simulink model "b0_loop"  (R2023b)
settings: Solver=FixedStepDiscrete  StartTime=0.0  StopTime=60  FixedStep=0.001  RelTol=1e-3
undefined symbols (not defined in the file or in its folder): DiscIntNeverNeededParam
settings Model: Creator=28447  LastModifiedBy=28447
settings SFSimCC: SimCustomHeaderCode=extern void b0_ident_sim(float iq, float u, float omega, float e1, float v, float *b0, float *du);  SimUserIncludeDirs=D:\Desktop\RCESO\simulink
settings SFSimCC: SimUserSources=|
  | D:\Desktop\RCESO\simulink\b0_ident.c
  | D:\Desktop\RCESO\simulink\b0_ident_wrap.c

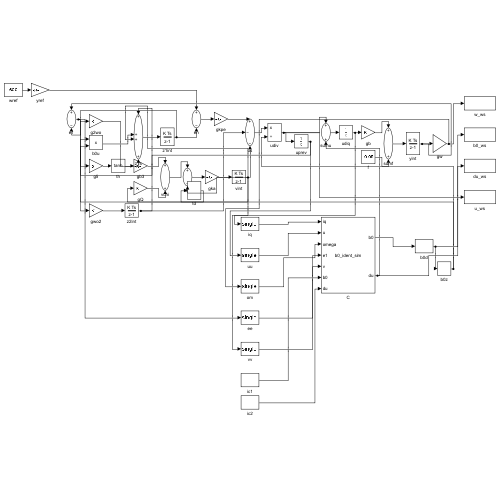
[thumbnail: Simulink's stored preview of the top-level diagram]
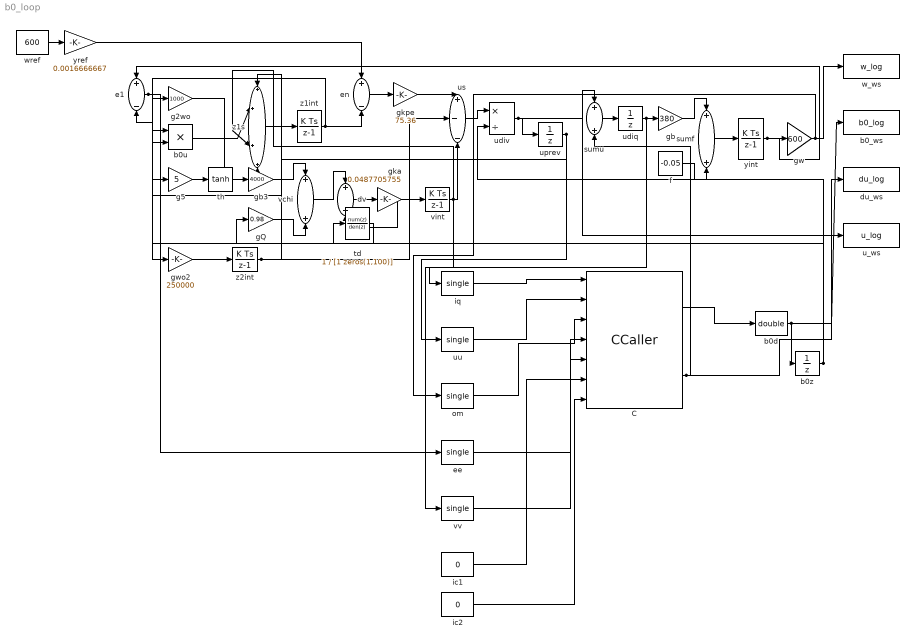
== system b0_loop ==
  C : CCaller  FunctionName=b0_ident_sim  PortSpecificationStruct="%)30     .    ^ L   8    (     @         %    \"     <    !     0         %  0 \"0    $    _    07)G3F%M90  4&]R=$YA;64 4V-O<&4     26YD97@     5'EP90      4VEZ90      27-';&]B86P   X    P    !@    @    $          4    (     0    (    !         !   @!I<0  #@   #     &    \"     0         !0    @    !     @    $         $  \" &EQ   .    .     8    (    !          %    \"     $    %     0         0  ...(+3754 chars)"
  b0_ws : ToWorkspace  VariableName=b0_log  SaveFormat=Timeseries  SampleTime=0.001
  b0d : DataTypeConversion  OutDataTypeStr=double  SaturateOnIntegerOverflow=off  RndMeth=Floor
  b0u : Product
  b0z : UnitDelay  InitialCondition=400  SampleTime=0.001  HasFrameUpgradeWarning=on
  du_ws : ToWorkspace  VariableName=du_log  SaveFormat=Timeseries  SampleTime=0.001
  dv : Sum  Inputs=+-
  e1 : Sum  Inputs=+-
  ee : DataTypeConversion  OutDataTypeStr=single  SaturateOnIntegerOverflow=off  RndMeth=Floor
  en : Sum  Inputs=+-
  f : Constant  Value=-0.05  SampleTime=0.001
  g2wo : Gain  Gain=1000
  g5 : Gain  Gain=5
  gQ : Gain  Gain=0.98
  gb : Gain  Gain=380
  gb3 : Gain  Gain=4000
  gka : Gain  Gain=0.0487705755
  gkpe : Gain  Gain=75.36
  gw : Gain  Gain=600
  gwo2 : Gain  Gain=250000
  ic1 : Constant  Value=0  OutDataTypeStr=single  SampleTime=0.001
  ic2 : Constant  Value=0  OutDataTypeStr=single  SampleTime=0.001
  iq : DataTypeConversion  OutDataTypeStr=single  SaturateOnIntegerOverflow=off  RndMeth=Floor
  om : DataTypeConversion  OutDataTypeStr=single  SaturateOnIntegerOverflow=off  RndMeth=Floor
  sumf : Sum
  sumu : Sum
  td : DiscreteTransferFcn  Numerator=1  Denominator=[1 zeros(1,100)]  SampleTime=0.001
  th : Trigonometry  Operator=tanh
  u_ws : ToWorkspace  VariableName=u_log  SaveFormat=Timeseries  SampleTime=0.001
  udiq : UnitDelay  SampleTime=0.001  HasFrameUpgradeWarning=on
  udiv : Product  Inputs=*/
  uprev : UnitDelay  SampleTime=0.001  HasFrameUpgradeWarning=on
  us : Sum  Inputs=+--
  uu : DataTypeConversion  OutDataTypeStr=single  SaturateOnIntegerOverflow=off  RndMeth=Floor
  vchi : Sum
  vint : DiscreteIntegrator  SampleTime=0.001  ICPrevOutput=DiscIntNeverNeededParam  ICPrevScaledInput=DiscIntNeverNeededParam
  vv : DataTypeConversion  OutDataTypeStr=single  SaturateOnIntegerOverflow=off  RndMeth=Floor
  w_ws : ToWorkspace  VariableName=w_log  SaveFormat=Timeseries  SampleTime=0.001
  wref : Constant  Value=600  SampleTime=0.001
  yint : DiscreteIntegrator  SampleTime=0.001  ICPrevOutput=DiscIntNeverNeededParam  ICPrevScaledInput=DiscIntNeverNeededParam
  yref : Gain  Gain=0.0016666667
  z1int : DiscreteIntegrator  SampleTime=0.001  ICPrevOutput=DiscIntNeverNeededParam  ICPrevScaledInput=DiscIntNeverNeededParam
  z1s : Sum  Inputs=++++
  z2int : DiscreteIntegrator  SampleTime=0.001  ICPrevOutput=DiscIntNeverNeededParam  ICPrevScaledInput=DiscIntNeverNeededParam
  wires:
  ic1/1 -> C/6
  ic2/1 -> C/7
  udiq/1 -> iq/1, gb/1
  iq/1 -> C/1
  uprev/1 -> uu/1, b0u/2
  uu/1 -> C/2
  gw/1 -> om/1, w_ws/1
  om/1 -> C/3
  e1/1 -> ee/1, g5/1, g2wo/1, gwo2/1
  ee/1 -> C/4
  vint/1 -> vv/1, td/1, dv/2, z1s/3, us/3
  vv/1 -> C/5
  C/1 -> b0d/1
  b0d/1 -> b0z/1, b0_ws/1
  wref/1 -> yref/1
  yint/1 -> e1/1, gw/1
  z1int/1 -> e1/2, en/2
  g5/1 -> th/1
  th/1 -> gb3/1
  td/1 -> gQ/1
  gb3/1 -> vchi/1
  gQ/1 -> vchi/2
  vchi/1 -> dv/1
  dv/1 -> gka/1
  gka/1 -> vint/1
  b0z/1 -> b0u/1, udiv/2
  z2int/1 -> z1s/1, us/2
  b0u/1 -> z1s/2
  g2wo/1 -> z1s/4
  z1s/1 -> z1int/1
  gwo2/1 -> z2int/1
  yref/1 -> en/1
  en/1 -> gkpe/1
  gkpe/1 -> us/1
  us/1 -> udiv/1
  udiv/1 -> uprev/1, sumu/1, u_ws/1
  C/2 -> sumu/2, du_ws/1
  sumu/1 -> udiq/1
  gb/1 -> sumf/1
  f/1 -> sumf/2
  sumf/1 -> yint/1
